simulink model "conveyor_belt_openloop"  (R2026a)
settings: Solver=ode4  StartTime=0  StopTime=20  FixedStep=0.01
PostLoadFcn:
  | mdlDir = fileparts(get_param('conveyor_belt_openloop', 'FileName'));
  | cadDir = fullfile(mdlDir, 'CAD');
  | addpath(cadDir);
  | prevDir = cd(cadDir);   % the copy in this folder wins over any other on the path
  | try
  |     convP = conveyor_belt_params();
  | catch paramsErr
  |     cd(prevDir); rethrow(paramsErr);
  | end
  | cd(prevDir);
  | missingFields = setdiff({'Ke', 'Tfric_Nm', 'bedFriction', 'beltDrag_N', 'beltTop_m', 'binFriction', 'contactOmega', 'contactZeta', 'controlPeriod_s', 'countsPerMotorRev', 'cycle_s', 'driverDrop_V', 'dropTimes_s', 'encWindow', 'frictionRate', 'g', 'gearEff', 'gearRatio', 'handOmega', 'handTime_s', 'itemFriction', 'itemMass_kg', 'itemSize_m', 'mmPerCount', 'motorR_ohm', 'rEff_m', 'restOffset_m', 'supplyV', 'vSlip', 'wSlip', 'xDrive_m', 'xDrop_m', 'xIdler_m', 'xReturn_m', 'zBinFloor_m', 'zCarry_m', 'zUnder_m', 'zWait_m'}, fieldnames(convP));
  | if ~isempty(missingFields)
  |     warning('Conveyor:params', '%s is older than this model (no %s). Replace it with the conveyor_belt_params.m that came with the model.', fullfile(cadDir, 'conveyor_belt_params.m'), strjoin(missingFields, ', '));
  | end
  | clear mdlDir cadDir prevDir missingFields
InitFcn:
  | mdlDir = fileparts(get_param('conveyor_belt_openloop', 'FileName'));
  | cadDir = fullfile(mdlDir, 'CAD');
  | addpath(cadDir);
  | prevDir = cd(cadDir);   % the copy in this folder wins over any other on the path
  | try
  |     convP = conveyor_belt_params();
  | catch paramsErr
  |     cd(prevDir); rethrow(paramsErr);
  | end
  | cd(prevDir);
  | missingFields = setdiff({'Ke', 'Tfric_Nm', 'bedFriction', 'beltDrag_N', 'beltTop_m', 'binFriction', 'contactOmega', 'contactZeta', 'controlPeriod_s', 'countsPerMotorRev', 'cycle_s', 'driverDrop_V', 'dropTimes_s', 'encWindow', 'frictionRate', 'g', 'gearEff', 'gearRatio', 'handOmega', 'handTime_s', 'itemFriction', 'itemMass_kg', 'itemSize_m', 'mmPerCount', 'motorR_ohm', 'rEff_m', 'restOffset_m', 'supplyV', 'vSlip', 'wSlip', 'xDrive_m', 'xDrop_m', 'xIdler_m', 'xReturn_m', 'zBinFloor_m', 'zCarry_m', 'zUnder_m', 'zWait_m'}, fieldnames(convP));
  | if isfield(convP, 'plaChain') && convP.plaChain ~= 0
  |     warning('Conveyor:belt', 'plaChain in conveyor_belt_params.m changed since this model was built: run build_conveyor_models so the 3-D parts match.');
  | end
  | if ~isempty(missingFields)
  |     error('Conveyor:params', '%s is older than this model (no %s). Replace it with the conveyor_belt_params.m that came with the model.', fullfile(cadDir, 'conveyor_belt_params.m'), strjoin(missingFields, ', '));
  | end
  | if ~strcmpi(pwd, mdlDir), cd(mdlDir); end   % STEP files are loaded as CAD/<part>.step
  | clear mdlDir cadDir prevDir missingFields
undefined symbols (not defined in the file or in its folder): X, Y, Z
libraries: sm_lib x73, nesl_utility x53, simulink x3, aerolibanimutils x1, slpidlib x1
(part 3 of 3)

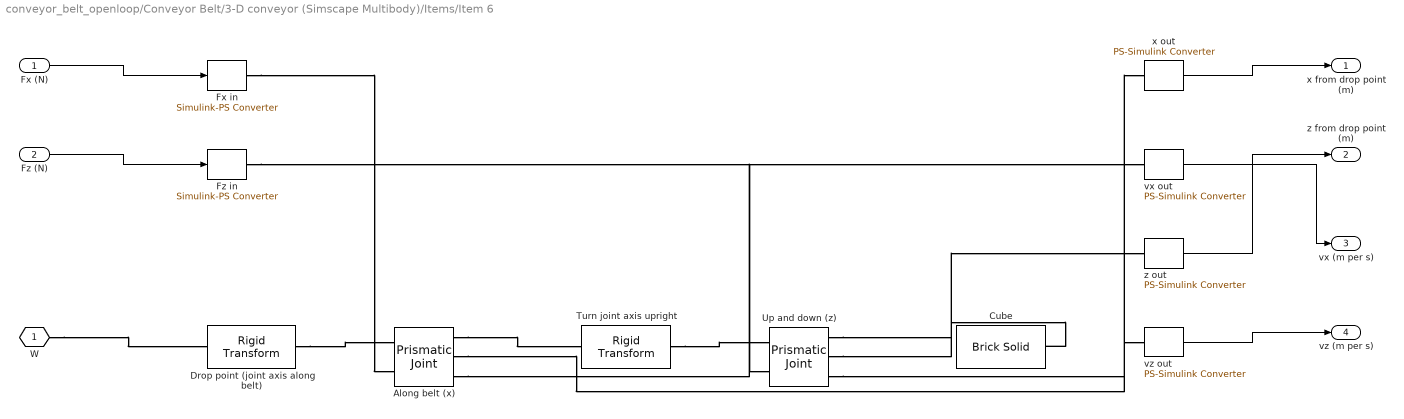
== system conveyor_belt_openloop/Conveyor Belt/3-D conveyor (Simscape Multibody)/Items/Item 6 ==
  Fx (N) : Inport
  Fz (N) : Inport  Port=2
  Along belt (x) : sm_lib/Joints/Prismatic Joint  JointMode=Normal  CompositeWrenchDir=FollowerOnBase  CompositeWrenchFrame=BaseFrame  SenseConstraintForce=off  SenseConstraintTorque=off  SenseTotalForce=off  SenseTotalTorque=off  PositionTargetSpecify=off  PositionTargetPriority=High  PositionTargetValue=0  PositionTargetValueUnits=m  VelocityTargetSpecify=off  VelocityTargetPriority=High  VelocityTargetValue=0  VelocityTargetValueUnits=m/s  EquilibriumPosition=0  EquilibriumPositionUnits=m  SpringStiffness=0  SpringStiffnessUnits=N/m  DampingCoefficient=0  DampingCoefficientUnits=N/(m/s)  LowerLimitSpecify=off  LowerLimitBound=-1  LowerLimitBoundUnits=m  LowerLimitStiffness=1e6  LowerLimitStiffnessUnits=N/m  LowerLimitDamping=1e3  LowerLimitDampingUnits=N/(m/s)  LowerLimitTransitionRegionWidth=1e-4  LowerLimitTransitionRegionWidthUnits=m  UpperLimitSpecify=off  UpperLimitBound=1  UpperLimitBoundUnits=m  UpperLimitStiffness=1e6  UpperLimitStiffnessUnits=N/m  UpperLimitDamping=1e3  UpperLimitDampingUnits=N/(m/s)  UpperLimitTransitionRegionWidth=1e-4  UpperLimitTransitionRegionWidthUnits=m  TorqueActuationMode=InputTorque  MotionActuationMode=ComputedMotion  SensePosition=on  SenseVelocity=on  SenseAcceleration=off  SenseTorqueForce=off  SenseLowerLimitTorqueForce=off  SenseUpperLimitTorqueForce=off
  Cube : sm_lib/Body Elements/Brick Solid  BrickDimensions=[1 1 1]*convP.itemSize_m  BrickDimensionsUnits=m  ExportEntireGeometry=off  InertiaType=CalculateFromGeometry  BasedOnType=Density  Density=convP.itemDensity_kgm3  DensityUnits=kg/m^3  Mass=1  MassUnits=kg  CenterOfMass=[0 0 0]  CenterOfMassUnits=m  MomentsOfInertia=[1 1 1]  MomentsOfInertiaUnits=kg*m^2  ProductsOfInertia=[0 0 0]  ProductsOfInertiaUnits=kg*m^2  GraphicType=FromGeometry  MarkerShape=Sphere  MarkerSize=10  GraphicVisPropType=SimpleVisualProperties  GraphicDiffuseColor=[0.9 0.25 0.25]  GraphicOpacity=1  GraphicSpecularColor=[0.5 0.5 0.5 1.0]  GraphicAmbientColor=[0.15 0.15 0.15 1.0]  GraphicEmissiveColor=[0.0 0.0 0.0 1.0]  GraphicShininess=75  DoExposeReferenceFrame=on  SerializedFrames=<Frames/>
  Drop point (joint axis along belt) : sm_lib/Frames and Transforms/Rigid Transform  RotationMethod=StandardAxis  FollAlignAxisA=+X  BaseAlignAxisA=+Y  FollAlignAxisB=+Y  BaseAlignAxisB=+Z  RotationStandardAxis=+Y  RotationAngle=90  RotationAngleUnits=deg  RotationArbitraryAxis=[0 0 1]  RotationSequenceAxes=FollowerAxes  RotationSequence=XYX  RotationSequenceAngles=[0 0 0]  RotationSequenceAnglesUnits=deg  RotationMatrix=[1 0 0;0 1 0;0 0 1]  Quaternion=[1 0 0 0]  TranslationMethod=Cartesian  TranslationCartesianOffset=[convP.xDrop_m 0 convP.zWait_m]  TranslationCartesianOffsetUnits=m  TranslationStandardAxis=+Z  TranslationStandardOffset=0  TranslationStandardOffsetUnits=m  TranslationROffset=0  TranslationROffsetUnits=m  TranslationThetaOffset=0  TranslationThetaOffsetUnits=deg  TranslationZOffset=0  TranslationZOffsetUnits=m
  Fx in : nesl_utility/Simulink-PS Converter  PhysicalDomain=network_engine_domain  SubClassName=ps_input  LeftPortType=input  RightPortType=output  PseudoPeriodic=off  Frequencies=[]  NoiseDistribution=none  NoiseParameters=[]  Unit=N  AffineConversion=off  FilteringAndDerivatives=provide  SimscapeFilterOrder=1  InputFilterTimeConstant=0.001  UdotUserProvided=0
  Fz in : nesl_utility/Simulink-PS Converter  PhysicalDomain=network_engine_domain  SubClassName=ps_input  LeftPortType=input  RightPortType=output  PseudoPeriodic=off  Frequencies=[]  NoiseDistribution=none  NoiseParameters=[]  Unit=N  AffineConversion=off  FilteringAndDerivatives=provide  SimscapeFilterOrder=1  InputFilterTimeConstant=0.001  UdotUserProvided=0
  Turn joint axis upright : sm_lib/Frames and Transforms/Rigid Transform  RotationMethod=StandardAxis  FollAlignAxisA=+X  BaseAlignAxisA=+Y  FollAlignAxisB=+Y  BaseAlignAxisB=+Z  RotationStandardAxis=+Y  RotationAngle=-90  RotationAngleUnits=deg  RotationArbitraryAxis=[0 0 1]  RotationSequenceAxes=FollowerAxes  RotationSequence=XYX  RotationSequenceAngles=[0 0 0]  RotationSequenceAnglesUnits=deg  RotationMatrix=[1 0 0;0 1 0;0 0 1]  Quaternion=[1 0 0 0]  TranslationMethod=None  TranslationCartesianOffset=[0 0 0]  TranslationCartesianOffsetUnits=m  TranslationStandardAxis=+Z  TranslationStandardOffset=0  TranslationStandardOffsetUnits=m  TranslationROffset=0  TranslationROffsetUnits=m  TranslationThetaOffset=0  TranslationThetaOffsetUnits=deg  TranslationZOffset=0  TranslationZOffsetUnits=m
  Up and down (z) : sm_lib/Joints/Prismatic Joint  JointMode=Normal  CompositeWrenchDir=FollowerOnBase  CompositeWrenchFrame=BaseFrame  SenseConstraintForce=off  SenseConstraintTorque=off  SenseTotalForce=off  SenseTotalTorque=off  PositionTargetSpecify=off  PositionTargetPriority=High  PositionTargetValue=0  PositionTargetValueUnits=m  VelocityTargetSpecify=off  VelocityTargetPriority=High  VelocityTargetValue=0  VelocityTargetValueUnits=m/s  EquilibriumPosition=0  EquilibriumPositionUnits=m  SpringStiffness=0  SpringStiffnessUnits=N/m  DampingCoefficient=0  DampingCoefficientUnits=N/(m/s)  LowerLimitSpecify=off  LowerLimitBound=-1  LowerLimitBoundUnits=m  LowerLimitStiffness=1e6  LowerLimitStiffnessUnits=N/m  LowerLimitDamping=1e3  LowerLimitDampingUnits=N/(m/s)  LowerLimitTransitionRegionWidth=1e-4  LowerLimitTransitionRegionWidthUnits=m  UpperLimitSpecify=off  UpperLimitBound=1  UpperLimitBoundUnits=m  UpperLimitStiffness=1e6  UpperLimitStiffnessUnits=N/m  UpperLimitDamping=1e3  UpperLimitDampingUnits=N/(m/s)  UpperLimitTransitionRegionWidth=1e-4  UpperLimitTransitionRegionWidthUnits=m  TorqueActuationMode=InputTorque  MotionActuationMode=ComputedMotion  SensePosition=on  SenseVelocity=on  SenseAcceleration=off  SenseTorqueForce=off  SenseLowerLimitTorqueForce=off  SenseUpperLimitTorqueForce=off
  vx out : nesl_utility/PS-Simulink Converter  PhysicalDomain=network_engine_domain  SubClassName=ps_output  LeftPortType=input  RightPortType=output  PseudoPeriodic=off  Frequencies=[]  VectorFormat=inherit  Unit=m/s  AffineConversion=off
  vz out : nesl_utility/PS-Simulink Converter  PhysicalDomain=network_engine_domain  SubClassName=ps_output  LeftPortType=input  RightPortType=output  PseudoPeriodic=off  Frequencies=[]  VectorFormat=inherit  Unit=m/s  AffineConversion=off
  x out : nesl_utility/PS-Simulink Converter  PhysicalDomain=network_engine_domain  SubClassName=ps_output  LeftPortType=input  RightPortType=output  PseudoPeriodic=off  Frequencies=[]  VectorFormat=inherit  Unit=m  AffineConversion=off
  z out : nesl_utility/PS-Simulink Converter  PhysicalDomain=network_engine_domain  SubClassName=ps_output  LeftPortType=input  RightPortType=output  PseudoPeriodic=off  Frequencies=[]  VectorFormat=inherit  Unit=m  AffineConversion=off
  W : PMIOPort  Side=Left
  x from drop point (m) : Outport
  z from drop point (m) : Outport  Port=2
  vx (m per s) : Outport  Port=3
  vz (m per s) : Outport  Port=4
  wires:
  Fx (N)/1 -> Fx in/1
  Fz (N)/1 -> Fz in/1
  x out/1 -> x from drop point (m)/1
  z out/1 -> z from drop point (m)/1
  vx out/1 -> vx (m per s)/1
  vz out/1 -> vz (m per s)/1
  connections:
  W/RConn1 -- Drop point (joint axis along belt)/LConn1
  Drop point (joint axis along belt)/RConn1 -- Along belt (x)/LConn1
  Fx in/RConn1 -- Along belt (x)/LConn2
  Along belt (x)/RConn1 -- Turn joint axis upright/LConn1
  Turn joint axis upright/RConn1 -- Up and down (z)/LConn1
  Fz in/RConn1 -- Up and down (z)/LConn2
  Up and down (z)/RConn1 -- Cube/RConn1
  Along belt (x)/RConn2 -- x out/LConn1
  Along belt (x)/RConn3 -- vx out/LConn1
  Up and down (z)/RConn2 -- z out/LConn1
  Up and down (z)/RConn3 -- vz out/LConn1

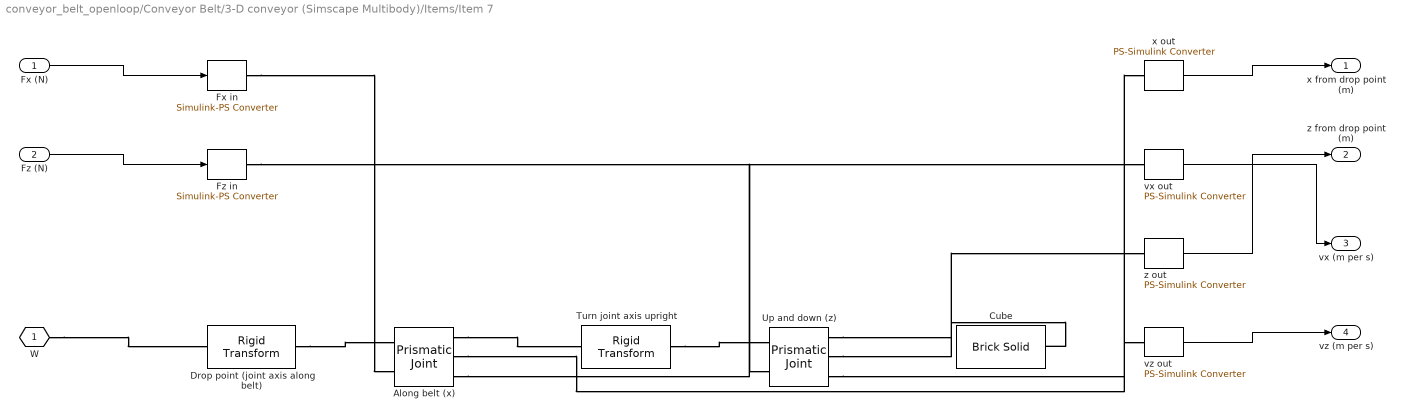
== system conveyor_belt_openloop/Conveyor Belt/3-D conveyor (Simscape Multibody)/Items/Item 7 ==
  Fx (N) : Inport
  Fz (N) : Inport  Port=2
  Along belt (x) : sm_lib/Joints/Prismatic Joint  JointMode=Normal  CompositeWrenchDir=FollowerOnBase  CompositeWrenchFrame=BaseFrame  SenseConstraintForce=off  SenseConstraintTorque=off  SenseTotalForce=off  SenseTotalTorque=off  PositionTargetSpecify=off  PositionTargetPriority=High  PositionTargetValue=0  PositionTargetValueUnits=m  VelocityTargetSpecify=off  VelocityTargetPriority=High  VelocityTargetValue=0  VelocityTargetValueUnits=m/s  EquilibriumPosition=0  EquilibriumPositionUnits=m  SpringStiffness=0  SpringStiffnessUnits=N/m  DampingCoefficient=0  DampingCoefficientUnits=N/(m/s)  LowerLimitSpecify=off  LowerLimitBound=-1  LowerLimitBoundUnits=m  LowerLimitStiffness=1e6  LowerLimitStiffnessUnits=N/m  LowerLimitDamping=1e3  LowerLimitDampingUnits=N/(m/s)  LowerLimitTransitionRegionWidth=1e-4  LowerLimitTransitionRegionWidthUnits=m  UpperLimitSpecify=off  UpperLimitBound=1  UpperLimitBoundUnits=m  UpperLimitStiffness=1e6  UpperLimitStiffnessUnits=N/m  UpperLimitDamping=1e3  UpperLimitDampingUnits=N/(m/s)  UpperLimitTransitionRegionWidth=1e-4  UpperLimitTransitionRegionWidthUnits=m  TorqueActuationMode=InputTorque  MotionActuationMode=ComputedMotion  SensePosition=on  SenseVelocity=on  SenseAcceleration=off  SenseTorqueForce=off  SenseLowerLimitTorqueForce=off  SenseUpperLimitTorqueForce=off
  Cube : sm_lib/Body Elements/Brick Solid  BrickDimensions=[1 1 1]*convP.itemSize_m  BrickDimensionsUnits=m  ExportEntireGeometry=off  InertiaType=CalculateFromGeometry  BasedOnType=Density  Density=convP.itemDensity_kgm3  DensityUnits=kg/m^3  Mass=1  MassUnits=kg  CenterOfMass=[0 0 0]  CenterOfMassUnits=m  MomentsOfInertia=[1 1 1]  MomentsOfInertiaUnits=kg*m^2  ProductsOfInertia=[0 0 0]  ProductsOfInertiaUnits=kg*m^2  GraphicType=FromGeometry  MarkerShape=Sphere  MarkerSize=10  GraphicVisPropType=SimpleVisualProperties  GraphicDiffuseColor=[0.9 0.25 0.25]  GraphicOpacity=1  GraphicSpecularColor=[0.5 0.5 0.5 1.0]  GraphicAmbientColor=[0.15 0.15 0.15 1.0]  GraphicEmissiveColor=[0.0 0.0 0.0 1.0]  GraphicShininess=75  DoExposeReferenceFrame=on  SerializedFrames=<Frames/>
  Drop point (joint axis along belt) : sm_lib/Frames and Transforms/Rigid Transform  RotationMethod=StandardAxis  FollAlignAxisA=+X  BaseAlignAxisA=+Y  FollAlignAxisB=+Y  BaseAlignAxisB=+Z  RotationStandardAxis=+Y  RotationAngle=90  RotationAngleUnits=deg  RotationArbitraryAxis=[0 0 1]  RotationSequenceAxes=FollowerAxes  RotationSequence=XYX  RotationSequenceAngles=[0 0 0]  RotationSequenceAnglesUnits=deg  RotationMatrix=[1 0 0;0 1 0;0 0 1]  Quaternion=[1 0 0 0]  TranslationMethod=Cartesian  TranslationCartesianOffset=[convP.xDrop_m 0 convP.zWait_m]  TranslationCartesianOffsetUnits=m  TranslationStandardAxis=+Z  TranslationStandardOffset=0  TranslationStandardOffsetUnits=m  TranslationROffset=0  TranslationROffsetUnits=m  TranslationThetaOffset=0  TranslationThetaOffsetUnits=deg  TranslationZOffset=0  TranslationZOffsetUnits=m
  Fx in : nesl_utility/Simulink-PS Converter  PhysicalDomain=network_engine_domain  SubClassName=ps_input  LeftPortType=input  RightPortType=output  PseudoPeriodic=off  Frequencies=[]  NoiseDistribution=none  NoiseParameters=[]  Unit=N  AffineConversion=off  FilteringAndDerivatives=provide  SimscapeFilterOrder=1  InputFilterTimeConstant=0.001  UdotUserProvided=0
  Fz in : nesl_utility/Simulink-PS Converter  PhysicalDomain=network_engine_domain  SubClassName=ps_input  LeftPortType=input  RightPortType=output  PseudoPeriodic=off  Frequencies=[]  NoiseDistribution=none  NoiseParameters=[]  Unit=N  AffineConversion=off  FilteringAndDerivatives=provide  SimscapeFilterOrder=1  InputFilterTimeConstant=0.001  UdotUserProvided=0
  Turn joint axis upright : sm_lib/Frames and Transforms/Rigid Transform  RotationMethod=StandardAxis  FollAlignAxisA=+X  BaseAlignAxisA=+Y  FollAlignAxisB=+Y  BaseAlignAxisB=+Z  RotationStandardAxis=+Y  RotationAngle=-90  RotationAngleUnits=deg  RotationArbitraryAxis=[0 0 1]  RotationSequenceAxes=FollowerAxes  RotationSequence=XYX  RotationSequenceAngles=[0 0 0]  RotationSequenceAnglesUnits=deg  RotationMatrix=[1 0 0;0 1 0;0 0 1]  Quaternion=[1 0 0 0]  TranslationMethod=None  TranslationCartesianOffset=[0 0 0]  TranslationCartesianOffsetUnits=m  TranslationStandardAxis=+Z  TranslationStandardOffset=0  TranslationStandardOffsetUnits=m  TranslationROffset=0  TranslationROffsetUnits=m  TranslationThetaOffset=0  TranslationThetaOffsetUnits=deg  TranslationZOffset=0  TranslationZOffsetUnits=m
  Up and down (z) : sm_lib/Joints/Prismatic Joint  JointMode=Normal  CompositeWrenchDir=FollowerOnBase  CompositeWrenchFrame=BaseFrame  SenseConstraintForce=off  SenseConstraintTorque=off  SenseTotalForce=off  SenseTotalTorque=off  PositionTargetSpecify=off  PositionTargetPriority=High  PositionTargetValue=0  PositionTargetValueUnits=m  VelocityTargetSpecify=off  VelocityTargetPriority=High  VelocityTargetValue=0  VelocityTargetValueUnits=m/s  EquilibriumPosition=0  EquilibriumPositionUnits=m  SpringStiffness=0  SpringStiffnessUnits=N/m  DampingCoefficient=0  DampingCoefficientUnits=N/(m/s)  LowerLimitSpecify=off  LowerLimitBound=-1  LowerLimitBoundUnits=m  LowerLimitStiffness=1e6  LowerLimitStiffnessUnits=N/m  LowerLimitDamping=1e3  LowerLimitDampingUnits=N/(m/s)  LowerLimitTransitionRegionWidth=1e-4  LowerLimitTransitionRegionWidthUnits=m  UpperLimitSpecify=off  UpperLimitBound=1  UpperLimitBoundUnits=m  UpperLimitStiffness=1e6  UpperLimitStiffnessUnits=N/m  UpperLimitDamping=1e3  UpperLimitDampingUnits=N/(m/s)  UpperLimitTransitionRegionWidth=1e-4  UpperLimitTransitionRegionWidthUnits=m  TorqueActuationMode=InputTorque  MotionActuationMode=ComputedMotion  SensePosition=on  SenseVelocity=on  SenseAcceleration=off  SenseTorqueForce=off  SenseLowerLimitTorqueForce=off  SenseUpperLimitTorqueForce=off
  vx out : nesl_utility/PS-Simulink Converter  PhysicalDomain=network_engine_domain  SubClassName=ps_output  LeftPortType=input  RightPortType=output  PseudoPeriodic=off  Frequencies=[]  VectorFormat=inherit  Unit=m/s  AffineConversion=off
  vz out : nesl_utility/PS-Simulink Converter  PhysicalDomain=network_engine_domain  SubClassName=ps_output  LeftPortType=input  RightPortType=output  PseudoPeriodic=off  Frequencies=[]  VectorFormat=inherit  Unit=m/s  AffineConversion=off
  x out : nesl_utility/PS-Simulink Converter  PhysicalDomain=network_engine_domain  SubClassName=ps_output  LeftPortType=input  RightPortType=output  PseudoPeriodic=off  Frequencies=[]  VectorFormat=inherit  Unit=m  AffineConversion=off
  z out : nesl_utility/PS-Simulink Converter  PhysicalDomain=network_engine_domain  SubClassName=ps_output  LeftPortType=input  RightPortType=output  PseudoPeriodic=off  Frequencies=[]  VectorFormat=inherit  Unit=m  AffineConversion=off
  W : PMIOPort  Side=Left
  x from drop point (m) : Outport
  z from drop point (m) : Outport  Port=2
  vx (m per s) : Outport  Port=3
  vz (m per s) : Outport  Port=4
  wires:
  Fx (N)/1 -> Fx in/1
  Fz (N)/1 -> Fz in/1
  x out/1 -> x from drop point (m)/1
  z out/1 -> z from drop point (m)/1
  vx out/1 -> vx (m per s)/1
  vz out/1 -> vz (m per s)/1
  connections:
  W/RConn1 -- Drop point (joint axis along belt)/LConn1
  Drop point (joint axis along belt)/RConn1 -- Along belt (x)/LConn1
  Fx in/RConn1 -- Along belt (x)/LConn2
  Along belt (x)/RConn1 -- Turn joint axis upright/LConn1
  Turn joint axis upright/RConn1 -- Up and down (z)/LConn1
  Fz in/RConn1 -- Up and down (z)/LConn2
  Up and down (z)/RConn1 -- Cube/RConn1
  Along belt (x)/RConn2 -- x out/LConn1
  Along belt (x)/RConn3 -- vx out/LConn1
  Up and down (z)/RConn2 -- z out/LConn1
  Up and down (z)/RConn3 -- vz out/LConn1

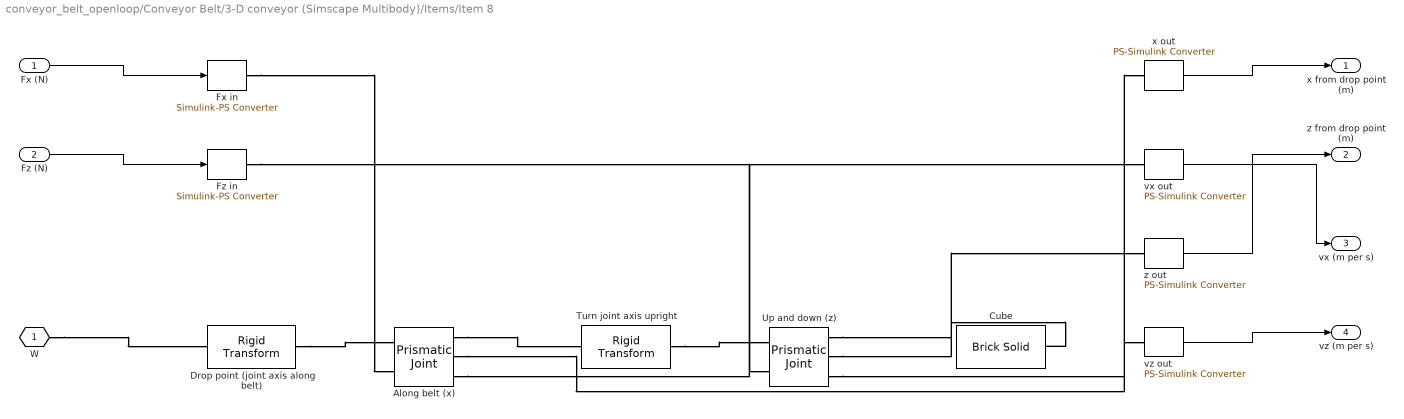
== system conveyor_belt_openloop/Conveyor Belt/3-D conveyor (Simscape Multibody)/Items/Item 8 ==
  Fx (N) : Inport
  Fz (N) : Inport  Port=2
  Along belt (x) : sm_lib/Joints/Prismatic Joint  JointMode=Normal  CompositeWrenchDir=FollowerOnBase  CompositeWrenchFrame=BaseFrame  SenseConstraintForce=off  SenseConstraintTorque=off  SenseTotalForce=off  SenseTotalTorque=off  PositionTargetSpecify=off  PositionTargetPriority=High  PositionTargetValue=0  PositionTargetValueUnits=m  VelocityTargetSpecify=off  VelocityTargetPriority=High  VelocityTargetValue=0  VelocityTargetValueUnits=m/s  EquilibriumPosition=0  EquilibriumPositionUnits=m  SpringStiffness=0  SpringStiffnessUnits=N/m  DampingCoefficient=0  DampingCoefficientUnits=N/(m/s)  LowerLimitSpecify=off  LowerLimitBound=-1  LowerLimitBoundUnits=m  LowerLimitStiffness=1e6  LowerLimitStiffnessUnits=N/m  LowerLimitDamping=1e3  LowerLimitDampingUnits=N/(m/s)  LowerLimitTransitionRegionWidth=1e-4  LowerLimitTransitionRegionWidthUnits=m  UpperLimitSpecify=off  UpperLimitBound=1  UpperLimitBoundUnits=m  UpperLimitStiffness=1e6  UpperLimitStiffnessUnits=N/m  UpperLimitDamping=1e3  UpperLimitDampingUnits=N/(m/s)  UpperLimitTransitionRegionWidth=1e-4  UpperLimitTransitionRegionWidthUnits=m  TorqueActuationMode=InputTorque  MotionActuationMode=ComputedMotion  SensePosition=on  SenseVelocity=on  SenseAcceleration=off  SenseTorqueForce=off  SenseLowerLimitTorqueForce=off  SenseUpperLimitTorqueForce=off
  Cube : sm_lib/Body Elements/Brick Solid  BrickDimensions=[1 1 1]*convP.itemSize_m  BrickDimensionsUnits=m  ExportEntireGeometry=off  InertiaType=CalculateFromGeometry  BasedOnType=Density  Density=convP.itemDensity_kgm3  DensityUnits=kg/m^3  Mass=1  MassUnits=kg  CenterOfMass=[0 0 0]  CenterOfMassUnits=m  MomentsOfInertia=[1 1 1]  MomentsOfInertiaUnits=kg*m^2  ProductsOfInertia=[0 0 0]  ProductsOfInertiaUnits=kg*m^2  GraphicType=FromGeometry  MarkerShape=Sphere  MarkerSize=10  GraphicVisPropType=SimpleVisualProperties  GraphicDiffuseColor=[0.9 0.25 0.25]  GraphicOpacity=1  GraphicSpecularColor=[0.5 0.5 0.5 1.0]  GraphicAmbientColor=[0.15 0.15 0.15 1.0]  GraphicEmissiveColor=[0.0 0.0 0.0 1.0]  GraphicShininess=75  DoExposeReferenceFrame=on  SerializedFrames=<Frames/>
  Drop point (joint axis along belt) : sm_lib/Frames and Transforms/Rigid Transform  RotationMethod=StandardAxis  FollAlignAxisA=+X  BaseAlignAxisA=+Y  FollAlignAxisB=+Y  BaseAlignAxisB=+Z  RotationStandardAxis=+Y  RotationAngle=90  RotationAngleUnits=deg  RotationArbitraryAxis=[0 0 1]  RotationSequenceAxes=FollowerAxes  RotationSequence=XYX  RotationSequenceAngles=[0 0 0]  RotationSequenceAnglesUnits=deg  RotationMatrix=[1 0 0;0 1 0;0 0 1]  Quaternion=[1 0 0 0]  TranslationMethod=Cartesian  TranslationCartesianOffset=[convP.xDrop_m 0 convP.zWait_m]  TranslationCartesianOffsetUnits=m  TranslationStandardAxis=+Z  TranslationStandardOffset=0  TranslationStandardOffsetUnits=m  TranslationROffset=0  TranslationROffsetUnits=m  TranslationThetaOffset=0  TranslationThetaOffsetUnits=deg  TranslationZOffset=0  TranslationZOffsetUnits=m
  Fx in : nesl_utility/Simulink-PS Converter  PhysicalDomain=network_engine_domain  SubClassName=ps_input  LeftPortType=input  RightPortType=output  PseudoPeriodic=off  Frequencies=[]  NoiseDistribution=none  NoiseParameters=[]  Unit=N  AffineConversion=off  FilteringAndDerivatives=provide  SimscapeFilterOrder=1  InputFilterTimeConstant=0.001  UdotUserProvided=0
  Fz in : nesl_utility/Simulink-PS Converter  PhysicalDomain=network_engine_domain  SubClassName=ps_input  LeftPortType=input  RightPortType=output  PseudoPeriodic=off  Frequencies=[]  NoiseDistribution=none  NoiseParameters=[]  Unit=N  AffineConversion=off  FilteringAndDerivatives=provide  SimscapeFilterOrder=1  InputFilterTimeConstant=0.001  UdotUserProvided=0
  Turn joint axis upright : sm_lib/Frames and Transforms/Rigid Transform  RotationMethod=StandardAxis  FollAlignAxisA=+X  BaseAlignAxisA=+Y  FollAlignAxisB=+Y  BaseAlignAxisB=+Z  RotationStandardAxis=+Y  RotationAngle=-90  RotationAngleUnits=deg  RotationArbitraryAxis=[0 0 1]  RotationSequenceAxes=FollowerAxes  RotationSequence=XYX  RotationSequenceAngles=[0 0 0]  RotationSequenceAnglesUnits=deg  RotationMatrix=[1 0 0;0 1 0;0 0 1]  Quaternion=[1 0 0 0]  TranslationMethod=None  TranslationCartesianOffset=[0 0 0]  TranslationCartesianOffsetUnits=m  TranslationStandardAxis=+Z  TranslationStandardOffset=0  TranslationStandardOffsetUnits=m  TranslationROffset=0  TranslationROffsetUnits=m  TranslationThetaOffset=0  TranslationThetaOffsetUnits=deg  TranslationZOffset=0  TranslationZOffsetUnits=m
  Up and down (z) : sm_lib/Joints/Prismatic Joint  JointMode=Normal  CompositeWrenchDir=FollowerOnBase  CompositeWrenchFrame=BaseFrame  SenseConstraintForce=off  SenseConstraintTorque=off  SenseTotalForce=off  SenseTotalTorque=off  PositionTargetSpecify=off  PositionTargetPriority=High  PositionTargetValue=0  PositionTargetValueUnits=m  VelocityTargetSpecify=off  VelocityTargetPriority=High  VelocityTargetValue=0  VelocityTargetValueUnits=m/s  EquilibriumPosition=0  EquilibriumPositionUnits=m  SpringStiffness=0  SpringStiffnessUnits=N/m  DampingCoefficient=0  DampingCoefficientUnits=N/(m/s)  LowerLimitSpecify=off  LowerLimitBound=-1  LowerLimitBoundUnits=m  LowerLimitStiffness=1e6  LowerLimitStiffnessUnits=N/m  LowerLimitDamping=1e3  LowerLimitDampingUnits=N/(m/s)  LowerLimitTransitionRegionWidth=1e-4  LowerLimitTransitionRegionWidthUnits=m  UpperLimitSpecify=off  UpperLimitBound=1  UpperLimitBoundUnits=m  UpperLimitStiffness=1e6  UpperLimitStiffnessUnits=N/m  UpperLimitDamping=1e3  UpperLimitDampingUnits=N/(m/s)  UpperLimitTransitionRegionWidth=1e-4  UpperLimitTransitionRegionWidthUnits=m  TorqueActuationMode=InputTorque  MotionActuationMode=ComputedMotion  SensePosition=on  SenseVelocity=on  SenseAcceleration=off  SenseTorqueForce=off  SenseLowerLimitTorqueForce=off  SenseUpperLimitTorqueForce=off
  vx out : nesl_utility/PS-Simulink Converter  PhysicalDomain=network_engine_domain  SubClassName=ps_output  LeftPortType=input  RightPortType=output  PseudoPeriodic=off  Frequencies=[]  VectorFormat=inherit  Unit=m/s  AffineConversion=off
  vz out : nesl_utility/PS-Simulink Converter  PhysicalDomain=network_engine_domain  SubClassName=ps_output  LeftPortType=input  RightPortType=output  PseudoPeriodic=off  Frequencies=[]  VectorFormat=inherit  Unit=m/s  AffineConversion=off
  x out : nesl_utility/PS-Simulink Converter  PhysicalDomain=network_engine_domain  SubClassName=ps_output  LeftPortType=input  RightPortType=output  PseudoPeriodic=off  Frequencies=[]  VectorFormat=inherit  Unit=m  AffineConversion=off
  z out : nesl_utility/PS-Simulink Converter  PhysicalDomain=network_engine_domain  SubClassName=ps_output  LeftPortType=input  RightPortType=output  PseudoPeriodic=off  Frequencies=[]  VectorFormat=inherit  Unit=m  AffineConversion=off
  W : PMIOPort  Side=Left
  x from drop point (m) : Outport
  z from drop point (m) : Outport  Port=2
  vx (m per s) : Outport  Port=3
  vz (m per s) : Outport  Port=4
  wires:
  Fx (N)/1 -> Fx in/1
  Fz (N)/1 -> Fz in/1
  x out/1 -> x from drop point (m)/1
  z out/1 -> z from drop point (m)/1
  vx out/1 -> vx (m per s)/1
  vz out/1 -> vz (m per s)/1
  connections:
  W/RConn1 -- Drop point (joint axis along belt)/LConn1
  Drop point (joint axis along belt)/RConn1 -- Along belt (x)/LConn1
  Fx in/RConn1 -- Along belt (x)/LConn2
  Along belt (x)/RConn1 -- Turn joint axis upright/LConn1
  Turn joint axis upright/RConn1 -- Up and down (z)/LConn1
  Fz in/RConn1 -- Up and down (z)/LConn2
  Up and down (z)/RConn1 -- Cube/RConn1
  Along belt (x)/RConn2 -- x out/LConn1
  Along belt (x)/RConn3 -- vx out/LConn1
  Up and down (z)/RConn2 -- z out/LConn1
  Up and down (z)/RConn3 -- vz out/LConn1

== matlab function conveyor_belt_openloop/Conveyor Belt/3-D conveyor (Simscape Multibody)/Belt and item contact ==
  data: px input; Fx output; pz input; vx input; vz input; vBelt input; tNow input; Fz output; Fload output; convP parameter
function [Fx, Fz, Fload] = beltContact(px, pz, vx, vz, vBelt, tNow, convP)
% Forces between each item and the belt (or the bin), and the load on the belt.
% Every item is dropped once per cycle. In the last second of its cycle it is
% returned to the chute, mostly hidden under the table, so 8 items last all run.
P = convP;
x = P.xDrop_m + px;  z = P.zWait_m + pz;     % joint positions -> world positions
n = numel(px);  Fx = zeros(n, 1);  Fz = zeros(n, 1);
h = P.itemSize_m;  m = P.itemMass_kg;
k = m*P.contactOmega^2;  c = 2*P.contactZeta*m*P.contactOmega;   % soft enough for ode4 at 10 ms
kh = m*P.handOmega^2;    ch = 2*m*P.handOmega;
Fitems = 0;  Nbelt = 0;
for q = 1:n
    tRel = tNow - P.dropTimes_s(q);
    if tRel < 0
        Fz(q) = m*P.g;                         % still in your hand
        continue
    end
    tc = mod(tRel, P.cycle_s);
    if tc > P.cycle_s - P.handTime_s           % being carried back to the chute
        s = (tc - (P.cycle_s - P.handTime_s))/P.handTime_s;
        if s < 0.2,       xT = x(q);        zT = P.zUnder_m;   % sink through the bin floor, out of sight
        elseif s < 0.45,  xT = P.xReturn_m; zT = P.zUnder_m;   % slide under the table
        elseif s < 0.7,   xT = P.xReturn_m; zT = P.zCarry_m;   % pop up just upstream of the conveyor
        elseif s < 0.85,  xT = P.xDrop_m;   zT = P.zCarry_m;   % over the top of the chute
        else,             xT = P.xDrop_m;   zT = P.zWait_m;    % down into the chute
        end
        Fx(q) = kh*(xT - x(q)) - ch*vx(q);
        Fz(q) = kh*(zT - z(q)) - ch*vz(q) + m*P.g;
        continue
    end
    if x(q) >= P.xIdler_m && x(q) <= P.xDrive_m
        pen = P.beltTop_m + h/2 + P.restOffset_m - z(q);   % how far it presses into the belt
        if pen > 0
            N = max(0, k*pen - c*vz(q));
            Fb = m*P.frictionRate*(vBelt - vx(q));          % belt drags item toward belt speed...
            Fb = min(max(Fb, -P.itemFriction*N), P.itemFriction*N);   % ...but no more than friction allows
            Fx(q) = Fb;  Fz(q) = N;  Fitems = Fitems + Fb;  Nbelt = Nbelt + N;
        end
    elseif x(q) > P.xDrive_m
        pen = P.zBinFloor_m + h/2 + P.restOffset_m - z(q);  % fell off the end into the bin
        if pen > 0
            N = max(0, k*pen - c*vz(q));
            Ff = -m*P.frictionRate*vx(q);
            Fx(q) = min(max(Ff, -P.binFriction*N), P.binFriction*N);  Fz(q) = N;
        end
    end
end
Fload = Fitems + (P.beltDrag_N + P.bedFriction*Nbelt)*tanh(vBelt/P.vSlip);
end

== matlab function conveyor_belt_openloop/Conveyor Belt/Actuator (driver + gearmotor)/DC motor and gearbox ==
  data: Vcmd input; Fpull output; wRoller input; current output; Vmotor output; convP parameter
function [Fpull, current, Vmotor] = motorGearbox(Vcmd, wRoller, convP)
% Arduino PWM -> logic-level MOSFET -> 12 V gearmotor (TS25GA) -> straight into the drive roller.
P = convP;
Vpwm   = round(Vcmd/P.supplyV*255)/255*P.supplyV;     % analogWrite() has 256 steps
Vmotor = Vpwm*(P.supplyV - P.driverDrop_V)/P.supplyV;  % volts actually across the motor
wMotor = P.gearRatio*wRoller;                          % motor shaft spins gearRatio (10) x faster
current = (Vmotor - P.Ke*wMotor)/P.motorR_ohm;         % back-EMF opposes the supply
current = max(current, 0);   % flyback diode: the driver can push, it cannot brake
Tmotor = P.gearEff*P.Ke*current - P.Tfric_Nm*tanh(wMotor/P.wSlip);
Fpull  = Tmotor*P.gearRatio/P.rEff_m;                  % torque at the roller -> belt pull
end

== matlab function conveyor_belt_openloop/Conveyor Belt/Encoder (Hall, on the motor shaft)/Hall encoder count ==
  data: angle_rad input; count output; jitter_counts input; convP parameter
function count  = hallCount(angle_rad, jitter_counts, convP)
% The running count of encoder edges the Arduino has seen (a long int that keeps growing).
P = convP;
motorTurns = P.gearRatio*angle_rad/(2*pi);         % the encoder is on the motor shaft
count = floor(motorTurns*P.countsPerMotorRev + jitter_counts);
end

== matlab function conveyor_belt_openloop/Conveyor Belt/Arduino belt speed (encoder) ==
  data: count input; speed_mms output; convP parameter
function speed_mms  = arduinoBeltSpeed(count, convP)

P = convP;
persistent buf nRead
if isempty(buf)
    buf = zeros(1, 41); nRead = 0;
end
buf = [count, buf(1:end-1)];                        % newest first
nRead = min(nRead + 1, 1000);
W = P.encWindow;
if nRead > W
    speed_mms = (buf(1) - buf(W + 1))*P.mmPerCount/(W*P.controlPeriod_s);
else
    speed_mms = 0;
end
end
